simulink library "xps_library"  (Simulink 8.2)
settings: Solver=ode45  SolverMode=SingleTasking  StartTime=0.0  StopTime=10.0  RelTol=1e-3
undefined symbols (not defined in the file): sys_clk
libraries: xbsIndex_r4 x865, dspsigops x81, simulink x68, casper_library_flow_control x68, xps_library x25, casper_library_misc x4
(part 9 of 10)

== system xps_library/ADCs/adc_mkid_4x/conv1 ==
  In1 : Inport
  Concat : xbsIndex_r4/Concat  num_inputs=2  dbl_ovrd=off  block_type=concat
      settings: block_version=8.2.02
  Inverter : xbsIndex_r4/Inverter  en=off  latency=0  dbl_ovrd=off  block_type=inv
      settings: xl_area=[0, 0, 0, 0, 0, 0, 0]  block_version=8.2.02
  Reinterpret : xbsIndex_r4/Reinterpret  force_arith_type=on  arith_type="Signed  (2's comp)"  force_bin_pt=on  bin_pt=11  block_type=reinterpret
      settings: infoedit="Changes signal type without altering the binary representation.   You can changed the signal between signed and unsigned, and relocate the binary point.<P><P>Hardware notes: In hardware this block costs nothing.<P><P>Example:  Suppose the input is 6 bits wide, signed, with 2 fractional bits, and the output is forced to unsigned with 0 fractional bits.  Then an input of -2.0 (1110.00 in binary 2's complement) becomes an output of 56 (111000 in binary)."  block_version=8.2.02
  Slice : xbsIndex_r4/Slice  nbits=1  boolean_output=off  mode=Upper Bit Location + Width  bit1=0  base1=MSB of Input  bit0=0  base0=LSB of Input  dbl_ovrd=off  block_type=slice
      settings: infoedit="Extracts a given range of bits from each input sample and presents it at the output.  The output type is ordinarily unsigned with binary point at zero, but can be Boolean when the slice is one bit wide.<P><P>Hardware notes: In hardware this block costs nothing."  block_version=8.2.02
  Slice1 : xbsIndex_r4/Slice  nbits=11  boolean_output=off  mode=Lower Bit Location + Width  bit1=0  base1=MSB of Input  bit0=0  base0=LSB of Input  dbl_ovrd=off  block_type=slice
      settings: infoedit="Extracts a given range of bits from each input sample and presents it at the output.  The output type is ordinarily unsigned with binary point at zero, but can be Boolean when the slice is one bit wide.<P><P>Hardware notes: In hardware this block costs nothing."  block_version=8.2.02
  Out1 : Outport
  wires:
  In1/1 -> Slice1/1, Slice/1
  Slice/1 -> Inverter/1
  Inverter/1 -> Concat/1
  Slice1/1 -> Concat/2
  Concat/1 -> Reinterpret/1
  Reinterpret/1 -> Out1/1

== system xps_library/ADCs/adc_mkid_4x/conv2 ==
  In1 : Inport
  Concat : xbsIndex_r4/Concat  num_inputs=2  dbl_ovrd=off  block_type=concat
      settings: block_version=8.2.02
  Inverter : xbsIndex_r4/Inverter  en=off  latency=0  dbl_ovrd=off  block_type=inv
      settings: xl_area=[0, 0, 0, 0, 0, 0, 0]  block_version=8.2.02
  Reinterpret : xbsIndex_r4/Reinterpret  force_arith_type=on  arith_type="Signed  (2's comp)"  force_bin_pt=on  bin_pt=11  block_type=reinterpret
      settings: infoedit="Changes signal type without altering the binary representation.   You can changed the signal between signed and unsigned, and relocate the binary point.<P><P>Hardware notes: In hardware this block costs nothing.<P><P>Example:  Suppose the input is 6 bits wide, signed, with 2 fractional bits, and the output is forced to unsigned with 0 fractional bits.  Then an input of -2.0 (1110.00 in binary 2's complement) becomes an output of 56 (111000 in binary)."  block_version=8.2.02
  Slice : xbsIndex_r4/Slice  nbits=1  boolean_output=off  mode=Upper Bit Location + Width  bit1=0  base1=MSB of Input  bit0=0  base0=LSB of Input  dbl_ovrd=off  block_type=slice
      settings: infoedit="Extracts a given range of bits from each input sample and presents it at the output.  The output type is ordinarily unsigned with binary point at zero, but can be Boolean when the slice is one bit wide.<P><P>Hardware notes: In hardware this block costs nothing."  block_version=8.2.02
  Slice1 : xbsIndex_r4/Slice  nbits=11  boolean_output=off  mode=Lower Bit Location + Width  bit1=0  base1=MSB of Input  bit0=0  base0=LSB of Input  dbl_ovrd=off  block_type=slice
      settings: infoedit="Extracts a given range of bits from each input sample and presents it at the output.  The output type is ordinarily unsigned with binary point at zero, but can be Boolean when the slice is one bit wide.<P><P>Hardware notes: In hardware this block costs nothing."  block_version=8.2.02
  Out1 : Outport
  wires:
  In1/1 -> Slice1/1, Slice/1
  Slice/1 -> Inverter/1
  Inverter/1 -> Concat/1
  Slice1/1 -> Concat/2
  Concat/1 -> Reinterpret/1
  Reinterpret/1 -> Out1/1

== system xps_library/ADCs/adc_mkid_4x/conv3 ==
  In1 : Inport
  Concat : xbsIndex_r4/Concat  num_inputs=2  dbl_ovrd=off  block_type=concat
      settings: block_version=8.2.02
  Inverter : xbsIndex_r4/Inverter  en=off  latency=0  dbl_ovrd=off  block_type=inv
      settings: xl_area=[0, 0, 0, 0, 0, 0, 0]  block_version=8.2.02
  Reinterpret : xbsIndex_r4/Reinterpret  force_arith_type=on  arith_type="Signed  (2's comp)"  force_bin_pt=on  bin_pt=11  block_type=reinterpret
      settings: infoedit="Changes signal type without altering the binary representation.   You can changed the signal between signed and unsigned, and relocate the binary point.<P><P>Hardware notes: In hardware this block costs nothing.<P><P>Example:  Suppose the input is 6 bits wide, signed, with 2 fractional bits, and the output is forced to unsigned with 0 fractional bits.  Then an input of -2.0 (1110.00 in binary 2's complement) becomes an output of 56 (111000 in binary)."  block_version=8.2.02
  Slice : xbsIndex_r4/Slice  nbits=1  boolean_output=off  mode=Upper Bit Location + Width  bit1=0  base1=MSB of Input  bit0=0  base0=LSB of Input  dbl_ovrd=off  block_type=slice
      settings: infoedit="Extracts a given range of bits from each input sample and presents it at the output.  The output type is ordinarily unsigned with binary point at zero, but can be Boolean when the slice is one bit wide.<P><P>Hardware notes: In hardware this block costs nothing."  block_version=8.2.02
  Slice1 : xbsIndex_r4/Slice  nbits=11  boolean_output=off  mode=Lower Bit Location + Width  bit1=0  base1=MSB of Input  bit0=0  base0=LSB of Input  dbl_ovrd=off  block_type=slice
      settings: infoedit="Extracts a given range of bits from each input sample and presents it at the output.  The output type is ordinarily unsigned with binary point at zero, but can be Boolean when the slice is one bit wide.<P><P>Hardware notes: In hardware this block costs nothing."  block_version=8.2.02
  Out1 : Outport
  wires:
  Reinterpret/1 -> Out1/1
  Concat/1 -> Reinterpret/1
  Slice1/1 -> Concat/2
  Inverter/1 -> Concat/1
  Slice/1 -> Inverter/1
  In1/1 -> Slice/1, Slice1/1

== system xps_library/ADCs/adc_mkid_4x/conv4 ==
  In1 : Inport
  Concat : xbsIndex_r4/Concat  num_inputs=2  dbl_ovrd=off  block_type=concat
      settings: block_version=8.2.02
  Inverter : xbsIndex_r4/Inverter  en=off  latency=0  dbl_ovrd=off  block_type=inv
      settings: xl_area=[0, 0, 0, 0, 0, 0, 0]  block_version=8.2.02
  Reinterpret : xbsIndex_r4/Reinterpret  force_arith_type=on  arith_type="Signed  (2's comp)"  force_bin_pt=on  bin_pt=11  block_type=reinterpret
      settings: infoedit="Changes signal type without altering the binary representation.   You can changed the signal between signed and unsigned, and relocate the binary point.<P><P>Hardware notes: In hardware this block costs nothing.<P><P>Example:  Suppose the input is 6 bits wide, signed, with 2 fractional bits, and the output is forced to unsigned with 0 fractional bits.  Then an input of -2.0 (1110.00 in binary 2's complement) becomes an output of 56 (111000 in binary)."  block_version=8.2.02
  Slice : xbsIndex_r4/Slice  nbits=1  boolean_output=off  mode=Upper Bit Location + Width  bit1=0  base1=MSB of Input  bit0=0  base0=LSB of Input  dbl_ovrd=off  block_type=slice
      settings: infoedit="Extracts a given range of bits from each input sample and presents it at the output.  The output type is ordinarily unsigned with binary point at zero, but can be Boolean when the slice is one bit wide.<P><P>Hardware notes: In hardware this block costs nothing."  block_version=8.2.02
  Slice1 : xbsIndex_r4/Slice  nbits=11  boolean_output=off  mode=Lower Bit Location + Width  bit1=0  base1=MSB of Input  bit0=0  base0=LSB of Input  dbl_ovrd=off  block_type=slice
      settings: infoedit="Extracts a given range of bits from each input sample and presents it at the output.  The output type is ordinarily unsigned with binary point at zero, but can be Boolean when the slice is one bit wide.<P><P>Hardware notes: In hardware this block costs nothing."  block_version=8.2.02
  Out1 : Outport
  wires:
  Reinterpret/1 -> Out1/1
  Concat/1 -> Reinterpret/1
  Slice1/1 -> Concat/2
  Inverter/1 -> Concat/1
  Slice/1 -> Inverter/1
  In1/1 -> Slice/1, Slice1/1

== system xps_library/ADCs/adc_mkid_4x/conv5 ==
  In1 : Inport
  Concat : xbsIndex_r4/Concat  num_inputs=2  dbl_ovrd=off  block_type=concat
      settings: block_version=8.2.02
  Inverter : xbsIndex_r4/Inverter  en=off  latency=0  dbl_ovrd=off  block_type=inv
      settings: xl_area=[0, 0, 0, 0, 0, 0, 0]  block_version=8.2.02
  Reinterpret : xbsIndex_r4/Reinterpret  force_arith_type=on  arith_type="Signed  (2's comp)"  force_bin_pt=on  bin_pt=11  block_type=reinterpret
      settings: infoedit="Changes signal type without altering the binary representation.   You can changed the signal between signed and unsigned, and relocate the binary point.<P><P>Hardware notes: In hardware this block costs nothing.<P><P>Example:  Suppose the input is 6 bits wide, signed, with 2 fractional bits, and the output is forced to unsigned with 0 fractional bits.  Then an input of -2.0 (1110.00 in binary 2's complement) becomes an output of 56 (111000 in binary)."  block_version=8.2.02
  Slice : xbsIndex_r4/Slice  nbits=1  boolean_output=off  mode=Upper Bit Location + Width  bit1=0  base1=MSB of Input  bit0=0  base0=LSB of Input  dbl_ovrd=off  block_type=slice
      settings: infoedit="Extracts a given range of bits from each input sample and presents it at the output.  The output type is ordinarily unsigned with binary point at zero, but can be Boolean when the slice is one bit wide.<P><P>Hardware notes: In hardware this block costs nothing."  block_version=8.2.02
  Slice1 : xbsIndex_r4/Slice  nbits=11  boolean_output=off  mode=Lower Bit Location + Width  bit1=0  base1=MSB of Input  bit0=0  base0=LSB of Input  dbl_ovrd=off  block_type=slice
      settings: infoedit="Extracts a given range of bits from each input sample and presents it at the output.  The output type is ordinarily unsigned with binary point at zero, but can be Boolean when the slice is one bit wide.<P><P>Hardware notes: In hardware this block costs nothing."  block_version=8.2.02
  Out1 : Outport
  wires:
  In1/1 -> Slice1/1, Slice/1
  Slice/1 -> Inverter/1
  Inverter/1 -> Concat/1
  Slice1/1 -> Concat/2
  Concat/1 -> Reinterpret/1
  Reinterpret/1 -> Out1/1

== system xps_library/ADCs/adc_mkid_4x/conv6 ==
  In1 : Inport
  Concat : xbsIndex_r4/Concat  num_inputs=2  dbl_ovrd=off  block_type=concat
      settings: block_version=8.2.02
  Inverter : xbsIndex_r4/Inverter  en=off  latency=0  dbl_ovrd=off  block_type=inv
      settings: xl_area=[0, 0, 0, 0, 0, 0, 0]  block_version=8.2.02
  Reinterpret : xbsIndex_r4/Reinterpret  force_arith_type=on  arith_type="Signed  (2's comp)"  force_bin_pt=on  bin_pt=11  block_type=reinterpret
      settings: infoedit="Changes signal type without altering the binary representation.   You can changed the signal between signed and unsigned, and relocate the binary point.<P><P>Hardware notes: In hardware this block costs nothing.<P><P>Example:  Suppose the input is 6 bits wide, signed, with 2 fractional bits, and the output is forced to unsigned with 0 fractional bits.  Then an input of -2.0 (1110.00 in binary 2's complement) becomes an output of 56 (111000 in binary)."  block_version=8.2.02
  Slice : xbsIndex_r4/Slice  nbits=1  boolean_output=off  mode=Upper Bit Location + Width  bit1=0  base1=MSB of Input  bit0=0  base0=LSB of Input  dbl_ovrd=off  block_type=slice
      settings: infoedit="Extracts a given range of bits from each input sample and presents it at the output.  The output type is ordinarily unsigned with binary point at zero, but can be Boolean when the slice is one bit wide.<P><P>Hardware notes: In hardware this block costs nothing."  block_version=8.2.02
  Slice1 : xbsIndex_r4/Slice  nbits=11  boolean_output=off  mode=Lower Bit Location + Width  bit1=0  base1=MSB of Input  bit0=0  base0=LSB of Input  dbl_ovrd=off  block_type=slice
      settings: infoedit="Extracts a given range of bits from each input sample and presents it at the output.  The output type is ordinarily unsigned with binary point at zero, but can be Boolean when the slice is one bit wide.<P><P>Hardware notes: In hardware this block costs nothing."  block_version=8.2.02
  Out1 : Outport
  wires:
  In1/1 -> Slice1/1, Slice/1
  Slice/1 -> Inverter/1
  Inverter/1 -> Concat/1
  Slice1/1 -> Concat/2
  Concat/1 -> Reinterpret/1
  Reinterpret/1 -> Out1/1

== system xps_library/ADCs/adc_mkid_4x/conv7 ==
  In1 : Inport
  Concat : xbsIndex_r4/Concat  num_inputs=2  dbl_ovrd=off  block_type=concat
      settings: block_version=8.2.02
  Inverter : xbsIndex_r4/Inverter  en=off  latency=0  dbl_ovrd=off  block_type=inv
      settings: xl_area=[0, 0, 0, 0, 0, 0, 0]  block_version=8.2.02
  Reinterpret : xbsIndex_r4/Reinterpret  force_arith_type=on  arith_type="Signed  (2's comp)"  force_bin_pt=on  bin_pt=11  block_type=reinterpret
      settings: infoedit="Changes signal type without altering the binary representation.   You can changed the signal between signed and unsigned, and relocate the binary point.<P><P>Hardware notes: In hardware this block costs nothing.<P><P>Example:  Suppose the input is 6 bits wide, signed, with 2 fractional bits, and the output is forced to unsigned with 0 fractional bits.  Then an input of -2.0 (1110.00 in binary 2's complement) becomes an output of 56 (111000 in binary)."  block_version=8.2.02
  Slice : xbsIndex_r4/Slice  nbits=1  boolean_output=off  mode=Upper Bit Location + Width  bit1=0  base1=MSB of Input  bit0=0  base0=LSB of Input  dbl_ovrd=off  block_type=slice
      settings: infoedit="Extracts a given range of bits from each input sample and presents it at the output.  The output type is ordinarily unsigned with binary point at zero, but can be Boolean when the slice is one bit wide.<P><P>Hardware notes: In hardware this block costs nothing."  block_version=8.2.02
  Slice1 : xbsIndex_r4/Slice  nbits=11  boolean_output=off  mode=Lower Bit Location + Width  bit1=0  base1=MSB of Input  bit0=0  base0=LSB of Input  dbl_ovrd=off  block_type=slice
      settings: infoedit="Extracts a given range of bits from each input sample and presents it at the output.  The output type is ordinarily unsigned with binary point at zero, but can be Boolean when the slice is one bit wide.<P><P>Hardware notes: In hardware this block costs nothing."  block_version=8.2.02
  Out1 : Outport
  wires:
  In1/1 -> Slice1/1, Slice/1
  Slice/1 -> Inverter/1
  Inverter/1 -> Concat/1
  Slice1/1 -> Concat/2
  Concat/1 -> Reinterpret/1
  Reinterpret/1 -> Out1/1

== system xps_library/DACs/dac_mkid/Subsystem ==
  pDataIn : Inport
  start : Inport  Port=2
  Concat : xbsIndex_r4/Concat  num_inputs=3  dbl_ovrd=off  block_type=concat
      settings: block_version=10.1.3
  Constant3 : xbsIndex_r4/Constant  const=0  gui_display_data_type=Fixed-point  arith_type=Unsigned  n_bits=4  bin_pt=0  preci_type=Single  exp_width=8  frac_width=24  explicit_period=on  period=1  equ=P=C  opselect=C  inp2=PCIN>>17  opr=+  inp1=P  carry=CIN  dbl_ovrd=off  block_type=constant
  Constant4 : xbsIndex_r4/Constant  const=2^1+2^3+2^5  gui_display_data_type=Fixed-point  arith_type=Unsigned  n_bits=9  bin_pt=0  preci_type=Single  exp_width=8  frac_width=24  explicit_period=on  period=1  equ=P=C  opselect=C  inp2=PCIN>>17  opr=+  inp1=P  carry=CIN  dbl_ovrd=off  block_type=constant
  Constant8 : xbsIndex_r4/Constant  const=2^17-1  gui_display_data_type=Fixed-point  arith_type=Unsigned  n_bits=17  bin_pt=0  preci_type=Single  exp_width=8  frac_width=24  explicit_period=on  period=1  equ=P=C  opselect=C  inp2=PCIN>>17  opr=+  inp1=P  carry=CIN  dbl_ovrd=off  block_type=constant
  Counter : xbsIndex_r4/Counter  cnt_type=Free Running  cnt_to=2048  operation=Up  start_count=0  cnt_by_val=1  arith_type=Unsigned  n_bits=7  bin_pt=0  load_pin=off  rst=on  en=on  explicit_period=on  period=1  dbl_ovrd=off  use_behavioral_HDL=off  implementation=Fabric  use_rpm=off  block_type=counter
  Delay : xbsIndex_r4/Delay  rst=off  infoeditControl=Selection of Reset will increase slice count due to use of real FFs and instead of SRLs  en=off  latency=15  dbl_ovrd=off  reg_retiming=off  block_type=delay
  Delay1 : xbsIndex_r4/Delay  rst=off  infoeditControl=Selection of Reset will increase slice count due to use of real FFs and instead of SRLs  en=off  latency=15  dbl_ovrd=off  reg_retiming=off  block_type=delay
  Delay2 : xbsIndex_r4/Delay  rst=off  infoeditControl=Selection of Reset will increase slice count due to use of real FFs and instead of SRLs  en=off  latency=15  dbl_ovrd=off  reg_retiming=off  block_type=delay
  Inverter : xbsIndex_r4/Inverter  en=off  latency=0  dbl_ovrd=off  block_type=inv
  Slice1 : xbsIndex_r4/Slice  nbits=7  boolean_output=on  mode=Lower Bit Location + Width  bit1=0  base1=MSB of Input  bit0=0  base0=MSB of Input  dbl_ovrd=off  block_type=slice
      settings: infoedit="Extracts a given range of bits from each input sample and presents it at the output.  The output type is ordinarily unsigned with binary point at zero, but can be Boolean when the slice is one bit wide.<P><P>Hardware notes: In hardware this block costs nothing."  block_version=10.1.3
  parallel_to_serial_converter : Subsystem  mask(parallel_to_serial_converter){pin_width=17, sout_width=1}
      mask prompts: pin_width "Parallel Input Width"; sout_width "Serial Output Width"
      mask help:
      | This block takes as input a parallel bus of specified width.
      | When the load signal 'ld' is asserted, this data is broken into
      | pieces of width specified by the serial output width and
      | stored into different registers chained to form a shift register.
      | If the 'shift' input is subsequently asserted, the shift register
      | returns as output a new piece of data of width sout_width.  This data
      | is the next least significant piece of the original bus.  The converter
      | serializes SMALL ENDIAN.
      |
      | Note that the load operation automatically loads the least significant
      | bits into the register closest to the output, so the first 'shift'
      | assertion changes the data output from bits [sout_width-1:0] to
      | bits [2*sout_width-1:sout_width].
      mask init:
      | % parallel_to_serial_converter_init(gcb, ...
      | %     'pin_width', pin_width, ...
      | %     'sout_width', sout_width);
  parallel_to_serial_converter1 : Subsystem  mask(parallel_to_serial_converter){pin_width=17, sout_width=1}
      mask prompts: pin_width "Parallel Input Width"; sout_width "Serial Output Width"
      mask help:
      | This block takes as input a parallel bus of specified width.
      | When the load signal 'ld' is asserted, this data is broken into
      | pieces of width specified by the serial output width and
      | stored into different registers chained to form a shift register.
      | If the 'shift' input is subsequently asserted, the shift register
      | returns as output a new piece of data of width sout_width.  This data
      | is the next least significant piece of the original bus.  The converter
      | serializes SMALL ENDIAN.
      |
      | Note that the load operation automatically loads the least significant
      | bits into the register closest to the output, so the first 'shift'
      | assertion changes the data output from bits [sout_width-1:0] to
      | bits [2*sout_width-1:sout_width].
      mask init:
      | % parallel_to_serial_converter_init(gcb, ...
      | %     'pin_width', pin_width, ...
      | %     'sout_width', sout_width);
  posedge1 : Subsystem  Tag=Rising Edge Detector  mask(posedge){}
      mask help: Outputs true if a boolean input signal is true this clock and was false last clock.
      mask Help: eval('xlWeb([getenv(''MLIB_ROOT''), ''\doc\htmlblocks\sp_posedge\sp_posedge.html''])')
  posedge2 : Subsystem  Tag=Rising Edge Detector  mask(posedge){}
      mask help: Outputs true if a boolean input signal is true this clock and was false last clock.
      mask Help: eval('xlWeb([getenv(''MLIB_ROOT''), ''\doc\htmlblocks\sp_posedge\sp_posedge.html''])')
  posedge3 : Subsystem  Tag=Rising Edge Detector  mask(posedge){}
      mask help: Outputs true if a boolean input signal is true this clock and was false last clock.
      mask Help: eval('xlWeb([getenv(''MLIB_ROOT''), ''\doc\htmlblocks\sp_posedge\sp_posedge.html''])')
  sDataOut : Outport
  enableOut : Outport  Port=2
  sclk : Outport  Port=3
  wires:
  posedge1/1(Out) -> parallel_to_serial_converter1/2(ld), parallel_to_serial_converter/2(ld)
  Constant3/1 -> Concat/3
  Constant4/1 -> Concat/1
  Concat/1 -> parallel_to_serial_converter/1(pin)
  Counter/1 -> Slice1/1
  Slice1/1 -> posedge2/1(In), Delay2/1
  posedge2/1(Out) -> parallel_to_serial_converter1/3(shift), parallel_to_serial_converter/3(shift)
  Constant8/1 -> parallel_to_serial_converter1/1(pin)
  parallel_to_serial_converter1/1(sout) -> Inverter/1
  start/1 -> posedge1/1(In), posedge3/1(In), Counter/2
  pDataIn/1 -> Concat/2
  Delay/1 -> Delay1/1
  parallel_to_serial_converter/1(sout) -> sDataOut/1
  Delay1/1 -> sclk/1
  Delay2/1 -> Delay/1
  Inverter/1 -> enableOut/1
  posedge3/1(Out) -> Counter/1

== system xps_library/DACs/dac_mkid_4x/Subsystem ==
  pDataIn : Inport
  start : Inport  Port=2
  Concat : xbsIndex_r4/Concat  num_inputs=3  dbl_ovrd=off  block_type=concat
      settings: block_version=10.1.3
  Constant3 : xbsIndex_r4/Constant  const=0  gui_display_data_type=Fixed-point  arith_type=Unsigned  n_bits=4  bin_pt=0  preci_type=Single  exp_width=8  frac_width=24  explicit_period=on  period=1  equ=P=C  opselect=C  inp2=PCIN>>17  opr=+  inp1=P  carry=CIN  dbl_ovrd=off  block_type=constant
  Constant4 : xbsIndex_r4/Constant  const=2^1+2^3+2^5  gui_display_data_type=Fixed-point  arith_type=Unsigned  n_bits=9  bin_pt=0  preci_type=Single  exp_width=8  frac_width=24  explicit_period=on  period=1  equ=P=C  opselect=C  inp2=PCIN>>17  opr=+  inp1=P  carry=CIN  dbl_ovrd=off  block_type=constant
  Constant8 : xbsIndex_r4/Constant  const=2^17-1  gui_display_data_type=Fixed-point  arith_type=Unsigned  n_bits=17  bin_pt=0  preci_type=Single  exp_width=8  frac_width=24  explicit_period=on  period=1  equ=P=C  opselect=C  inp2=PCIN>>17  opr=+  inp1=P  carry=CIN  dbl_ovrd=off  block_type=constant
  Counter : xbsIndex_r4/Counter  cnt_type=Free Running  cnt_to=2048  operation=Up  start_count=0  cnt_by_val=1  arith_type=Unsigned  n_bits=7  bin_pt=0  load_pin=off  rst=on  en=on  explicit_period=on  period=1  dbl_ovrd=off  use_behavioral_HDL=off  implementation=Fabric  use_rpm=off  block_type=counter
  Delay : xbsIndex_r4/Delay  rst=off  infoeditControl=Selection of Reset will increase slice count due to use of real FFs and instead of SRLs  en=off  latency=15  dbl_ovrd=off  reg_retiming=off  block_type=delay
  Delay1 : xbsIndex_r4/Delay  rst=off  infoeditControl=Selection of Reset will increase slice count due to use of real FFs and instead of SRLs  en=off  latency=15  dbl_ovrd=off  reg_retiming=off  block_type=delay
  Delay2 : xbsIndex_r4/Delay  rst=off  infoeditControl=Selection of Reset will increase slice count due to use of real FFs and instead of SRLs  en=off  latency=15  dbl_ovrd=off  reg_retiming=off  block_type=delay
  Inverter : xbsIndex_r4/Inverter  en=off  latency=0  dbl_ovrd=off  block_type=inv
  Slice1 : xbsIndex_r4/Slice  nbits=7  boolean_output=on  mode=Lower Bit Location + Width  bit1=0  base1=MSB of Input  bit0=0  base0=MSB of Input  dbl_ovrd=off  block_type=slice
      settings: infoedit="Extracts a given range of bits from each input sample and presents it at the output.  The output type is ordinarily unsigned with binary point at zero, but can be Boolean when the slice is one bit wide.<P><P>Hardware notes: In hardware this block costs nothing."  block_version=10.1.3
  parallel_to_serial_converter : Subsystem  mask(parallel_to_serial_converter){pin_width=17, sout_width=1}
      mask prompts: pin_width "Parallel Input Width"; sout_width "Serial Output Width"
      mask help:
      | This block takes as input a parallel bus of specified width.
      | When the load signal 'ld' is asserted, this data is broken into
      | pieces of width specified by the serial output width and
      | stored into different registers chained to form a shift register.
      | If the 'shift' input is subsequently asserted, the shift register
      | returns as output a new piece of data of width sout_width.  This data
      | is the next least significant piece of the original bus.  The converter
      | serializes SMALL ENDIAN.
      |
      | Note that the load operation automatically loads the least significant
      | bits into the register closest to the output, so the first 'shift'
      | assertion changes the data output from bits [sout_width-1:0] to
      | bits [2*sout_width-1:sout_width].
      mask init:
      | %parallel_to_serial_converter_init(gcb, ...
      | %    'pin_width', pin_width, ...
      | %    'sout_width', sout_width);
  parallel_to_serial_converter1 : Subsystem  mask(parallel_to_serial_converter){pin_width=17, sout_width=1}
      mask prompts: pin_width "Parallel Input Width"; sout_width "Serial Output Width"
      mask help:
      | This block takes as input a parallel bus of specified width.
      | When the load signal 'ld' is asserted, this data is broken into
      | pieces of width specified by the serial output width and
      | stored into different registers chained to form a shift register.
      | If the 'shift' input is subsequently asserted, the shift register
      | returns as output a new piece of data of width sout_width.  This data
      | is the next least significant piece of the original bus.  The converter
      | serializes SMALL ENDIAN.
      |
      | Note that the load operation automatically loads the least significant
      | bits into the register closest to the output, so the first 'shift'
      | assertion changes the data output from bits [sout_width-1:0] to
      | bits [2*sout_width-1:sout_width].
      mask init:
      | % parallel_to_serial_converter_init(gcb, ...
      | %     'pin_width', pin_width, ...
      | %     'sout_width', sout_width);
  posedge1 : Subsystem  Tag=Rising Edge Detector  mask(posedge){}
      mask help: Outputs true if a boolean input signal is true this clock and was false last clock.
      mask Help: eval('xlWeb([getenv(''MLIB_ROOT''), ''\doc\htmlblocks\sp_posedge\sp_posedge.html''])')
  posedge2 : Subsystem  Tag=Rising Edge Detector  mask(posedge){}
      mask help: Outputs true if a boolean input signal is true this clock and was false last clock.
      mask Help: eval('xlWeb([getenv(''MLIB_ROOT''), ''\doc\htmlblocks\sp_posedge\sp_posedge.html''])')
  posedge3 : Subsystem  Tag=Rising Edge Detector  mask(posedge){}
      mask help: Outputs true if a boolean input signal is true this clock and was false last clock.
      mask Help: eval('xlWeb([getenv(''MLIB_ROOT''), ''\doc\htmlblocks\sp_posedge\sp_posedge.html''])')
  sDataOut : Outport
  enableOut : Outport  Port=2
  sclk : Outport  Port=3
  wires:
  posedge3/1(Out) -> Counter/1
  Inverter/1 -> enableOut/1
  Delay2/1 -> Delay/1
  Delay1/1 -> sclk/1
  parallel_to_serial_converter/1(sout) -> sDataOut/1
  Delay/1 -> Delay1/1
  pDataIn/1 -> Concat/2
  start/1 -> Counter/2, posedge3/1(In), posedge1/1(In)
  parallel_to_serial_converter1/1(sout) -> Inverter/1
  Constant8/1 -> parallel_to_serial_converter1/1(pin)
  posedge2/1(Out) -> parallel_to_serial_converter1/3(shift), parallel_to_serial_converter/3(shift)
  Slice1/1 -> Delay2/1, posedge2/1(In)
  Counter/1 -> Slice1/1
  Concat/1 -> parallel_to_serial_converter/1(pin)
  Constant4/1 -> Concat/1
  Constant3/1 -> Concat/3
  posedge1/1(Out) -> parallel_to_serial_converter1/2(ld), parallel_to_serial_converter/2(ld)

== system xps_library/Shared_BRAM/mem/calc_add ==
  note: If reading/writing words
      | smaller than 32 bits,
      | change address so
      | that addressing is
      | big endian instead of
      | little, otherwise
      | pass through
  note: Use behavioural HDL
      | so that gets optimised
      | to minimum logic
  in : Inport
  add_sub : xbsIndex_r4/AddSub  mode=Subtraction  use_carryin=off  use_carryout=off  en=off  latency=0  precision=User Defined  arith_type=Unsigned  n_bits=max(1, log2(32/data_width))  bin_pt=0  quantization=Truncate  overflow=Wrap  dbl_ovrd=off  use_behavioral_HDL=on  hw_selection=Fabric  pipelined=off  block_type=addsub
  concat : xbsIndex_r4/Concat  num_inputs=2  dbl_ovrd=off  block_type=concat
  const : xbsIndex_r4/Constant  const=max(0, 32/data_width-1)  gui_display_data_type=Fixed-point  arith_type=Unsigned  n_bits=max(1, log2(32/data_width))  bin_pt=0  preci_type=Single  exp_width=8  frac_width=24  explicit_period=on  period=sample_rate  equ=P=C  opselect=C  inp2=PCIN>>17  opr=+  inp1=P  carry=CIN  dbl_ovrd=off  block_type=constant
      settings: block_version=11.4
  convert_addr : xbsIndex_r4/Convert  gui_display_data_type=Fixed-point  arith_type=Unsigned  n_bits=addr_width  bin_pt=0  float_type=Single  exp_bits=8  fraction_bits=24  quantization=Truncate  overflow=Wrap  en=off  latency=0  dbl_ovrd=off  pipeline=off  block_type=convert
      settings: xl_area=[0, 0, 0, 0, 0, 0, 0]
  lsw : xbsIndex_r4/Slice  nbits=max(1, log2(32/data_width))  boolean_output=off  mode=Lower Bit Location + Width  bit1=0  base1=MSB of Input  bit0=0  base0=LSB of Input  dbl_ovrd=off  block_type=slice
  manipulate : xbsIndex_r4/Constant  const=min(1, floor(32/data_width) - 1)  gui_display_data_type=Fixed-point  arith_type=Unsigned  n_bits=1  bin_pt=0  preci_type=Single  exp_width=8  frac_width=24  explicit_period=on  period=sample_rate  equ=P=C  opselect=C  inp2=PCIN>>17  opr=+  inp1=P  carry=CIN  dbl_ovrd=off  block_type=constant
      settings: block_version=11.4
  msw : xbsIndex_r4/Slice  nbits=addr_width - max(1, log2(32/data_width))  boolean_output=off  mode=Upper Bit Location + Width  bit1=0  base1=MSB of Input  bit0=0  base0=LSB of Input  dbl_ovrd=off  block_type=slice
  mux : xbsIndex_r4/Mux  inputs=2  en=off  latency=0  precision=Full  arith_type=Unsigned  n_bits=16  bin_pt=14  quantization=Truncate  overflow=Wrap  dbl_ovrd=off  block_type=mux
      settings: block_version=11.4
  out : Outport
  wires:
  in/1 -> convert_addr/1
  add_sub/1 -> concat/2
  msw/1 -> concat/1
  concat/1 -> mux/3
  manipulate/1 -> mux/1
  mux/1 -> out/1
  lsw/1 -> add_sub/2
  const/1 -> add_sub/1
  convert_addr/1 -> lsw/1, msw/1, mux/2

== system xps_library/Shared_BRAM/mem/sim_munge_in ==
  din : Inport
  reinterpret_out : xbsIndex_r4/Reinterpret  force_arith_type=on  arith_type=Unsigned  force_bin_pt=on  bin_pt=0  block_type=reinterpret
  dout : Outport
  wires:
  din/1 -> reinterpret_out/1
  reinterpret_out/1 -> dout/1

== system xps_library/Shared_BRAM/mem/sim_munge_out ==
  din : Inport
  reinterpret_out : xbsIndex_r4/Reinterpret  force_arith_type=on  arith_type=Unsigned  force_bin_pt=on  bin_pt=0  block_type=reinterpret
  dout : Outport
  wires:
  din/1 -> reinterpret_out/1
  reinterpret_out/1 -> dout/1

== system xps_library/dram/dram_sim/memory ==
  addr : Inport
  wren : Inport  Port=2
  wrbe : Inport  Port=3
  wrdata : Inport  Port=4
  rden : Inport  Port=5
  Delay : xbsIndex_r4/Delay  rst=off  infoeditControl=Selection of Reset will increase slice count due to use of real FFs and instead of SRLs  en=off  latency=1  dbl_ovrd=off  reg_retiming=off  block_type=delay
  Delay1 : xbsIndex_r4/Delay  rst=off  infoeditControl=Selection of Reset will increase slice count due to use of real FFs and instead of SRLs  en=off  latency=7  dbl_ovrd=off  reg_retiming=off  block_type=delay
  Delay2 : xbsIndex_r4/Delay  rst=off  infoeditControl=Selection of Reset will increase slice count due to use of real FFs and instead of SRLs  en=off  latency=7  dbl_ovrd=off  reg_retiming=off  block_type=delay
  Disregard Subsystem : xbsIndex_r4/Disregard Subsystem  Tag=discardX  block_type=disregard
  cast_narrow1 : xbsIndex_r4/Convert  gui_display_data_type=Fixed-point  arith_type=Unsigned  n_bits=36  bin_pt=0  float_type=Single  exp_bits=8  fraction_bits=24  quantization=Truncate  overflow=Wrap  en=off  latency=0  dbl_ovrd=off  pipeline=off  block_type=convert
      settings: xl_area=[0, 0, 0, 0, 0, 0, 0]
  cast_narrow2 : xbsIndex_r4/Convert  gui_display_data_type=Fixed-point  arith_type=Unsigned  n_bits=288  bin_pt=0  float_type=Single  exp_bits=8  fraction_bits=24  quantization=Truncate  overflow=Wrap  en=off  latency=0  dbl_ovrd=off  pipeline=off  block_type=convert
      settings: xl_area=[0, 0, 0, 0, 0, 0, 0]
  cast_narrow3 : xbsIndex_r4/Convert  gui_display_data_type=Fixed-point  arith_type=Unsigned  n_bits=288  bin_pt=0  float_type=Single  exp_bits=8  fraction_bits=24  quantization=Truncate  overflow=Wrap  en=off  latency=0  dbl_ovrd=off  pipeline=off  block_type=convert
      settings: xl_area=[0, 0, 0, 0, 0, 0, 0]
  cast_narrow4 : xbsIndex_r4/Convert  gui_display_data_type=Fixed-point  arith_type=Unsigned  n_bits=ram_depth  bin_pt=0  float_type=Single  exp_bits=8  fraction_bits=24  quantization=Truncate  overflow=Wrap  en=off  latency=0  dbl_ovrd=off  pipeline=off  block_type=convert
      settings: xl_area=[0, 0, 0, 0, 0, 0, 0]
  ram0 : xbsIndex_r4/Single Port RAM  depth=2^ram_depth  initVector=sin(pi*(0:15)/2^ram_depth)  distributed_mem=Block RAM  write_mode=Read After Write  rst=off  init_reg=0  en=off  latency=1  dbl_ovrd=off  optimize=Area  block_type=spram
      settings: block_version=10.1.3
  rddata : Outport
  rdvld : Outport  Port=2
  wires:
  wrdata/1 -> cast_narrow2/1
  wrbe/1 -> cast_narrow1/1
  addr/1 -> cast_narrow4/1
  cast_narrow1/1 -> [b]
  wren/1 -> ram0/3
  cast_narrow2/1 -> ram0/2
  rden/1 -> Delay/1
  Delay/1 -> Delay1/1
  Delay2/1 -> cast_narrow3/1
  Delay1/1 -> rdvld/1
  cast_narrow3/1 -> rddata/1
  ram0/1 -> Delay2/1
  cast_narrow4/1 -> ram0/1

== system xps_library/dram/dram_sim/rd_sm ==
  rd_ack : Inport
  rst : Inport  Port=2
  fifo_empty : Inport  Port=3
  Constant : xbsIndex_r4/Constant  const=0  gui_display_data_type=Fixed-point  arith_type=Unsigned  n_bits=2  bin_pt=0  preci_type=Single  exp_width=8  frac_width=24  explicit_period=off  period=1  equ=P=C  opselect=C  inp2=PCIN>>17  opr=+  inp1=P  carry=CIN  dbl_ovrd=off  block_type=constant
  Constant{1,4..5,8} (4 alike) : xbsIndex_r4/Constant  const=1  gui_display_data_type=Fixed-point  arith_type=Unsigned  n_bits=2  bin_pt=0  preci_type=Single  exp_width=8  frac_width=24  explicit_period=off  period=1  equ=P=C  opselect=C  inp2=PCIN>>17  opr=+  inp1=P  carry=CIN  dbl_ovrd=off  block_type=constant
  Constant2 : xbsIndex_r4/Constant  const=2  gui_display_data_type=Fixed-point  arith_type=Unsigned  n_bits=2  bin_pt=0  preci_type=Single  exp_width=8  frac_width=24  explicit_period=off  period=1  equ=P=C  opselect=C  inp2=PCIN>>17  opr=+  inp1=P  carry=CIN  dbl_ovrd=off  block_type=constant
  Constant3 : xbsIndex_r4/Constant  const=0  gui_display_data_type=Fixed-point  arith_type=Unsigned  n_bits=2  bin_pt=0  preci_type=Single  exp_width=8  frac_width=24  explicit_period=off  period=1  equ=P=C  opselect=C  inp2=PCIN>>17  opr=+  inp1=P  carry=CIN  dbl_ovrd=off  block_type=constant
  Constant6 : xbsIndex_r4/Constant  const=2  gui_display_data_type=Fixed-point  arith_type=Unsigned  n_bits=2  bin_pt=0  preci_type=Single  exp_width=8  frac_width=24  explicit_period=off  period=1  equ=P=C  opselect=C  inp2=PCIN>>17  opr=+  inp1=P  carry=CIN  dbl_ovrd=off  block_type=constant
  Constant7 : xbsIndex_r4/Constant  const=2  gui_display_data_type=Fixed-point  arith_type=Unsigned  n_bits=2  bin_pt=0  preci_type=Single  exp_width=8  frac_width=24  explicit_period=off  period=1  equ=P=C  opselect=C  inp2=PCIN>>17  opr=+  inp1=P  carry=CIN  dbl_ovrd=off  block_type=constant
  Constant9 : xbsIndex_r4/Constant  const=0  gui_display_data_type=Fixed-point  arith_type=Unsigned  n_bits=2  bin_pt=0  preci_type=Single  exp_width=8  frac_width=24  explicit_period=off  period=1  equ=P=C  opselect=C  inp2=PCIN>>17  opr=+  inp1=P  carry=CIN  dbl_ovrd=off  block_type=constant
  Inverter : xbsIndex_r4/Inverter  en=off  latency=0  dbl_ovrd=off  block_type=inv
  Mux : xbsIndex_r4/Mux  inputs=3  en=off  latency=0  precision=Full  arith_type=Unsigned  n_bits=16  bin_pt=14  quantization=Truncate  overflow=Wrap  dbl_ovrd=off  block_type=mux
  Mux{1..4} (4 alike) : xbsIndex_r4/Mux  inputs=2  en=off  latency=0  precision=Full  arith_type=Unsigned  n_bits=16  bin_pt=14  quantization=Truncate  overflow=Wrap  dbl_ovrd=off  block_type=mux
  Register : xbsIndex_r4/Register  init=0  rst=on  en=off  dbl_ovrd=off  block_type=register
  Relational : xbsIndex_r4/Relational  mode=a=b  en=off  latency=0  dbl_ovrd=off  block_type=relational
      settings: block_version=10.1.3
  Relational1 : xbsIndex_r4/Relational  mode=a=b  en=off  latency=0  dbl_ovrd=off  block_type=relational
      settings: block_version=10.1.3
  Relational2 : xbsIndex_r4/Relational  mode=a=b  en=off  latency=0  dbl_ovrd=off  block_type=relational
      settings: block_version=10.1.3
  empty : Outport
  d0 : Outport  Port=2
  d1 : Outport  Port=3
  wires:
  rst/1 -> Register/2
  Register/1 -> Relational2/2, Relational/2, Relational1/2, [S]
  Constant/1 -> Relational/1
  Constant1/1 -> Relational1/1
  Constant2/1 -> Relational2/1
  Relational/1 -> empty/1
  Relational1/1 -> d0/1
  Relational2/1 -> d1/1
  [S] -> Mux/1
  Mux/1 -> Register/1
  Mux1/1 -> Mux/2
  Constant3/1 -> Mux1/2
  Inverter/1 -> Mux1/1
  fifo_empty/1 -> Inverter/1, Mux4/1
  Constant4/1 -> Mux1/3
  Constant5/1 -> Mux2/2
  Constant6/1 -> Mux2/3
  Mux2/1 -> Mux/3
  rd_ack/1 -> Mux2/1, Mux3/1
  Mux3/1 -> Mux/4
  Constant7/1 -> Mux3/2
  Mux4/1 -> Mux3/3
  Constant8/1 -> Mux4/2
  Constant9/1 -> Mux4/3

== system xps_library/ADCs/adc083000x2/adc_sim/overflow_detector ==
  s0 : Inport
  s1 : Inport  Port=2
  s2 : Inport  Port=3
  s3 : Inport  Port=4
  s4 : Inport  Port=5
  s5 : Inport  Port=6
  s6 : Inport  Port=7
  s7 : Inport  Port=8
  s8 : Inport  Port=9
  s9 : Inport  Port=10
  s10 : Inport  Port=11
  s11 : Inport  Port=12
  s12 : Inport  Port=13
  s13 : Inport  Port=14
  s14 : Inport  Port=15
  s15 : Inport  Port=16
  Add : Sum  Inputs=++++++++
  of{0..6} (7 alike) : xps_library/ADCs/of1  bit_num=0  n_adc_bits=8
  of7 : casper_library_misc/of1  bit_num=0  n_adc_bits=8
  overflow : Outport
  wires:
  s0/1 -> of0/1
  s8/1 -> of0/2
  of0/1 -> Add/1
  s1/1 -> of1/1
  s9/1 -> of1/2
  of1/1 -> Add/2
  s2/1 -> of2/1
  s10/1 -> of2/2
  of2/1 -> Add/3
  s3/1 -> of3/1
  s11/1 -> of3/2
  of3/1 -> Add/4
  s4/1 -> of4/1
  s12/1 -> of4/2
  of4/1 -> Add/5
  s5/1 -> of5/1
  s13/1 -> of5/2
  of5/1 -> Add/6
  s6/1 -> of6/1
  s14/1 -> of6/2
  of6/1 -> Add/7

== system xps_library/DACs/dac_mkid/Subsystem/parallel_to_serial_converter ==
  pin : Inport
  ld : Inport  Port=2
  shift : Inport  Port=3
  Logical : xbsIndex_r4/Logical  logical_function=OR  inputs=2  en=off  latency=0  precision=Full  arith_type=Unsigned  n_bits=16  bin_pt=0  align_bp=on  dbl_ovrd=off  block_type=logical
  filler : xbsIndex_r4/Constant  const=0  gui_display_data_type=Fixed-point  arith_type=Unsigned  n_bits=sout_width  bin_pt=0  preci_type=Single  exp_width=8  frac_width=24  explicit_period=on  period=1  equ=P=C  opselect=C  inp2=PCIN>>17  opr=+  inp1=P  carry=CIN  dbl_ovrd=off  block_type=constant
  shifter_unit1 : casper_library_flow_control/shifter_unit  data_width=1  pin_offset=0
  shifter_unit10 : casper_library_flow_control/shifter_unit  data_width=1  pin_offset=9
  shifter_unit11 : casper_library_flow_control/shifter_unit  data_width=1  pin_offset=10
  shifter_unit12 : casper_library_flow_control/shifter_unit  data_width=1  pin_offset=11
  shifter_unit13 : casper_library_flow_control/shifter_unit  data_width=1  pin_offset=12
  shifter_unit14 : casper_library_flow_control/shifter_unit  data_width=1  pin_offset=13
  shifter_unit15 : casper_library_flow_control/shifter_unit  data_width=1  pin_offset=14
  shifter_unit16 : casper_library_flow_control/shifter_unit  data_width=1  pin_offset=15
  shifter_unit17 : casper_library_flow_control/shifter_unit  data_width=1  pin_offset=16
  shifter_unit2 : casper_library_flow_control/shifter_unit  data_width=1  pin_offset=1
  shifter_unit3 : casper_library_flow_control/shifter_unit  data_width=1  pin_offset=2
  shifter_unit4 : casper_library_flow_control/shifter_unit  data_width=1  pin_offset=3
  shifter_unit5 : casper_library_flow_control/shifter_unit  data_width=1  pin_offset=4
  shifter_unit6 : casper_library_flow_control/shifter_unit  data_width=1  pin_offset=5
  shifter_unit7 : casper_library_flow_control/shifter_unit  data_width=1  pin_offset=6
  shifter_unit8 : casper_library_flow_control/shifter_unit  data_width=1  pin_offset=7
  shifter_unit9 : casper_library_flow_control/shifter_unit  data_width=1  pin_offset=8
  sout : Outport
  wires:
  ld/1 -> Logical/1, shifter_unit1/1, shifter_unit2/1, shifter_unit3/1, shifter_unit4/1, shifter_unit5/1, shifter_unit6/1, shifter_unit7/1, shifter_unit8/1, shifter_unit9/1, shifter_unit10/1, shifter_unit11/1, shifter_unit12/1, shifter_unit13/1, shifter_unit14/1, shifter_unit15/1, shifter_unit16/1, shifter_unit17/1
  shift/1 -> Logical/2
  filler/1 -> shifter_unit1/2
  pin/1 -> shifter_unit1/3, shifter_unit2/3, shifter_unit3/3, shifter_unit4/3, shifter_unit5/3, shifter_unit6/3, shifter_unit7/3, shifter_unit8/3, shifter_unit9/3, shifter_unit10/3, shifter_unit11/3, shifter_unit12/3, shifter_unit13/3, shifter_unit14/3, shifter_unit15/3, shifter_unit16/3, shifter_unit17/3
  Logical/1 -> shifter_unit1/4, shifter_unit2/4, shifter_unit3/4, shifter_unit4/4, shifter_unit5/4, shifter_unit6/4, shifter_unit7/4, shifter_unit8/4, shifter_unit9/4, shifter_unit10/4, shifter_unit11/4, shifter_unit12/4, shifter_unit13/4, shifter_unit14/4, shifter_unit15/4, shifter_unit16/4, shifter_unit17/4
  shifter_unit1/1 -> shifter_unit2/2
  shifter_unit2/1 -> shifter_unit3/2
  shifter_unit3/1 -> shifter_unit4/2
  shifter_unit4/1 -> shifter_unit5/2
  shifter_unit5/1 -> shifter_unit6/2
  shifter_unit6/1 -> shifter_unit7/2
  shifter_unit7/1 -> shifter_unit8/2
  shifter_unit8/1 -> shifter_unit9/2
  shifter_unit9/1 -> shifter_unit10/2
  shifter_unit10/1 -> shifter_unit11/2
  shifter_unit11/1 -> shifter_unit12/2
  shifter_unit12/1 -> shifter_unit13/2
  shifter_unit13/1 -> shifter_unit14/2
  shifter_unit14/1 -> shifter_unit15/2
  shifter_unit15/1 -> shifter_unit16/2
  shifter_unit16/1 -> shifter_unit17/2
  shifter_unit17/1 -> sout/1

== system xps_library/DACs/dac_mkid/Subsystem/parallel_to_serial_converter1 ==
  pin : Inport
  ld : Inport  Port=2
  shift : Inport  Port=3
  Logical : xbsIndex_r4/Logical  logical_function=OR  inputs=2  en=off  latency=0  precision=Full  arith_type=Unsigned  n_bits=16  bin_pt=0  align_bp=on  dbl_ovrd=off  block_type=logical
  filler : xbsIndex_r4/Constant  const=0  gui_display_data_type=Fixed-point  arith_type=Unsigned  n_bits=sout_width  bin_pt=0  preci_type=Single  exp_width=8  frac_width=24  explicit_period=on  period=1  equ=P=C  opselect=C  inp2=PCIN>>17  opr=+  inp1=P  carry=CIN  dbl_ovrd=off  block_type=constant
  shifter_unit1 : casper_library_flow_control/shifter_unit  data_width=1  pin_offset=0
  shifter_unit10 : casper_library_flow_control/shifter_unit  data_width=1  pin_offset=9
  shifter_unit11 : casper_library_flow_control/shifter_unit  data_width=1  pin_offset=10
  shifter_unit12 : casper_library_flow_control/shifter_unit  data_width=1  pin_offset=11
  shifter_unit13 : casper_library_flow_control/shifter_unit  data_width=1  pin_offset=12
  shifter_unit14 : casper_library_flow_control/shifter_unit  data_width=1  pin_offset=13
  shifter_unit15 : casper_library_flow_control/shifter_unit  data_width=1  pin_offset=14
  shifter_unit16 : casper_library_flow_control/shifter_unit  data_width=1  pin_offset=15
  shifter_unit17 : casper_library_flow_control/shifter_unit  data_width=1  pin_offset=16
  shifter_unit2 : casper_library_flow_control/shifter_unit  data_width=1  pin_offset=1
  shifter_unit3 : casper_library_flow_control/shifter_unit  data_width=1  pin_offset=2
  shifter_unit4 : casper_library_flow_control/shifter_unit  data_width=1  pin_offset=3
  shifter_unit5 : casper_library_flow_control/shifter_unit  data_width=1  pin_offset=4
  shifter_unit6 : casper_library_flow_control/shifter_unit  data_width=1  pin_offset=5
  shifter_unit7 : casper_library_flow_control/shifter_unit  data_width=1  pin_offset=6
  shifter_unit8 : casper_library_flow_control/shifter_unit  data_width=1  pin_offset=7
  shifter_unit9 : casper_library_flow_control/shifter_unit  data_width=1  pin_offset=8
  sout : Outport
  wires:
  ld/1 -> Logical/1, shifter_unit1/1, shifter_unit2/1, shifter_unit3/1, shifter_unit4/1, shifter_unit5/1, shifter_unit6/1, shifter_unit7/1, shifter_unit8/1, shifter_unit9/1, shifter_unit10/1, shifter_unit11/1, shifter_unit12/1, shifter_unit13/1, shifter_unit14/1, shifter_unit15/1, shifter_unit16/1, shifter_unit17/1
  shift/1 -> Logical/2
  filler/1 -> shifter_unit1/2
  pin/1 -> shifter_unit1/3, shifter_unit2/3, shifter_unit3/3, shifter_unit4/3, shifter_unit5/3, shifter_unit6/3, shifter_unit7/3, shifter_unit8/3, shifter_unit9/3, shifter_unit10/3, shifter_unit11/3, shifter_unit12/3, shifter_unit13/3, shifter_unit14/3, shifter_unit15/3, shifter_unit16/3, shifter_unit17/3
  Logical/1 -> shifter_unit1/4, shifter_unit2/4, shifter_unit3/4, shifter_unit4/4, shifter_unit5/4, shifter_unit6/4, shifter_unit7/4, shifter_unit8/4, shifter_unit9/4, shifter_unit10/4, shifter_unit11/4, shifter_unit12/4, shifter_unit13/4, shifter_unit14/4, shifter_unit15/4, shifter_unit16/4, shifter_unit17/4
  shifter_unit1/1 -> shifter_unit2/2
  shifter_unit2/1 -> shifter_unit3/2
  shifter_unit3/1 -> shifter_unit4/2
  shifter_unit4/1 -> shifter_unit5/2
  shifter_unit5/1 -> shifter_unit6/2
  shifter_unit6/1 -> shifter_unit7/2
  shifter_unit7/1 -> shifter_unit8/2
  shifter_unit8/1 -> shifter_unit9/2
  shifter_unit9/1 -> shifter_unit10/2
  shifter_unit10/1 -> shifter_unit11/2
  shifter_unit11/1 -> shifter_unit12/2
  shifter_unit12/1 -> shifter_unit13/2
  shifter_unit13/1 -> shifter_unit14/2
  shifter_unit14/1 -> shifter_unit15/2
  shifter_unit15/1 -> shifter_unit16/2
  shifter_unit16/1 -> shifter_unit17/2
  shifter_unit17/1 -> sout/1

== system xps_library/DACs/dac_mkid/Subsystem/posedge1 ==
  In : Inport
  Delay : xbsIndex_r4/Delay  rst=off  infoeditControl=Selection of Reset will increase slice count due to use of real FFs and instead of SRLs  en=off  latency=1  dbl_ovrd=off  reg_retiming=off  block_type=delay
      settings: xl_area=[0, 0, 0, 0, 0, 0, 0]  block_version=9.1.01
  Inverter : xbsIndex_r4/Inverter  en=off  latency=0  dbl_ovrd=off  block_type=inv
      settings: xl_area=[0, 0, 0, 0, 0, 0, 0]  block_version=9.1.01
  Logical : xbsIndex_r4/Logical  logical_function=AND  inputs=2  en=off  latency=0  precision=Full  arith_type=Unsigned  n_bits=8  bin_pt=2  align_bp=on  dbl_ovrd=off  block_type=logical
      settings: xl_area=[0, 0, 0, 0, 0, 0, 0]  block_version=9.1.01
  Out : Outport
  wires:
  Delay/1 -> Inverter/1
  Inverter/1 -> Logical/1
  In/1 -> Delay/1, Logical/2
  Logical/1 -> Out/1

== system xps_library/DACs/dac_mkid/Subsystem/posedge2 ==
  In : Inport
  Delay : xbsIndex_r4/Delay  rst=off  infoeditControl=Selection of Reset will increase slice count due to use of real FFs and instead of SRLs  en=off  latency=1  dbl_ovrd=off  reg_retiming=off  block_type=delay
      settings: xl_area=[0, 0, 0, 0, 0, 0, 0]  block_version=9.1.01
  Inverter : xbsIndex_r4/Inverter  en=off  latency=0  dbl_ovrd=off  block_type=inv
      settings: xl_area=[0, 0, 0, 0, 0, 0, 0]  block_version=9.1.01
  Logical : xbsIndex_r4/Logical  logical_function=AND  inputs=2  en=off  latency=0  precision=Full  arith_type=Unsigned  n_bits=8  bin_pt=2  align_bp=on  dbl_ovrd=off  block_type=logical
      settings: xl_area=[0, 0, 0, 0, 0, 0, 0]  block_version=9.1.01
  Out : Outport
  wires:
  Delay/1 -> Inverter/1
  Inverter/1 -> Logical/1
  In/1 -> Delay/1, Logical/2
  Logical/1 -> Out/1

== system xps_library/DACs/dac_mkid/Subsystem/posedge3 ==
  In : Inport
  Delay : xbsIndex_r4/Delay  rst=off  infoeditControl=Selection of Reset will increase slice count due to use of real FFs and instead of SRLs  en=off  latency=1  dbl_ovrd=off  reg_retiming=off  block_type=delay
      settings: xl_area=[0, 0, 0, 0, 0, 0, 0]  block_version=9.1.01
  Inverter : xbsIndex_r4/Inverter  en=off  latency=0  dbl_ovrd=off  block_type=inv
      settings: xl_area=[0, 0, 0, 0, 0, 0, 0]  block_version=9.1.01
  Logical : xbsIndex_r4/Logical  logical_function=AND  inputs=2  en=off  latency=0  precision=Full  arith_type=Unsigned  n_bits=8  bin_pt=2  align_bp=on  dbl_ovrd=off  block_type=logical
      settings: xl_area=[0, 0, 0, 0, 0, 0, 0]  block_version=9.1.01
  Out : Outport
  wires:
  Delay/1 -> Inverter/1
  Inverter/1 -> Logical/1
  In/1 -> Delay/1, Logical/2
  Logical/1 -> Out/1
